simulink model "AcceleratationCore"  (R2024b)
settings: Solver=FixedStepDiscrete  StartTime=0.0  StopTime=inf  FixedStep=1  RelTol=1e-3
model workspace (MATLAB code in the model file):
  | B      = 64;  K = 11;  Cin = 3;
  | L      = 2^nextpow2(B+K-1);   LOG2L = log2(L);   LOG2B = log2(B);
  | NKEEP  = L/2 + 1;
  | LAT    = 307;                              % from FFT_core icon after Ctrl+D
  | W      = ceil((LAT - L + NKEEP + 1)/L);    % wait frames
  | NFR    = B + W + NKEEP;                    % frames per channel
  | PH_W   = ceil(log2(NFR*L));   F_W = PH_W - LOG2L;
  | OC_MAX = (B + NKEEP)*L - 1;   OC_W = ceil(log2(OC_MAX + 1));
  | RAM_AW = LOG2B + LOG2L - 1;
  | WL_BUF = 16;
  | root = fileparts(get_param('AcceleratationCore', 'FileName'));            % repo root = first parent with "vectors"
  | while ~isfolder(fullfile(root, 'vectors')), up = fileparts(root); assert(~strcmp(up, root), 'Repo root not found.'); root = up; end
  | IMG = imresize(imread(fullfile(root, 'resources', 'fujian_mountain_227.png')), [227 227]);   % 227x227x3 uint8
  | Wk  = load(fullfile(root, 'vectors', 'phase1_inputs.mat'), 'W');
  | TILE = IMG(1:B, 1:B, 1);                       % first tile, R channel
  | P = zeros(ceil(size(IMG,1)/B)*B, ceil(size(IMG,2)/B)*B, 3, 'uint8');  P(1:size(IMG,1), 1:size(IMG,2), :) = IMG;
  | IMG_VEC = reshape(permute(reshape(P, B, size(P,1)/B, B, size(P,2)/B, 3), [3 1 5 4 2]), [], 1);   % tiles x Cin x B^2
  | TILE_VEC = reshape(TILE.', [], 1);             % row-major, as will send
  | Cout    = 2;                                   % first test, back to 96 after
  | X_WL    = 2*LOG2B + 8 + 1;                     % B*B*255 < 2^(X_WL-1)
  | KERN_WL = 16;                                  % kernel word (16-bit SDRAM)
  | ACC_WL  = X_WL + KERN_WL + 1 + ceil(log2(Cin));
  | TILE3_VEC = reshape(permute(IMG(1:B, 1:B, :), [2 1 3]), [], 1);   % 3 channels, row-major
  | Hk = fft2(rot90(Wk.W(:, :, :, 1:Cout), 2), L, L) / 255;          % Phase 1 method, 1/255 folded
  | Hk = Hk(:, 1:NKEEP, :, :);                                       % Hermitian half
  | s  = KERN_WL - 2 - floor(log2(max(abs([real(Hk(:)); imag(Hk(:))]))));
  | KERN_TAB = int16(round(reshape(permute(Hk, [3 1 2 4]), Cin, []) * 2^s));
  | IF_WL = 18;   % ifft2d datapath word length (18x18 DSP mode)
  | D_IN  = 16;   % measured 15 on fujian tile 1 (Cout 96) + 1 bit margin; saturation guards outliers
  | D_MID = 4;    % measured 3 + 1 bit margin
  | clear Wk
libraries: hdlsllib x5
settings Model: SimulationMode=accelerator  NumberOfSteps=100  Creator=aaala  LastModifiedBy=aaala
settings OptimizationCC: BlockReduction=off  ConditionallyExecuteInputs=off  DefaultParameterBehavior=Inlined
settings DebuggingCC: AlgebraicLoopMsg=error  InheritedTsInSrcMsg=error
settings HardwareCC: ProdBitPerPointer=32  ProdBitPerSizeT=32  ProdBitPerPtrDiffT=32  ProdLargestAtomicFloat=None  ProdIntDivRoundTo=Undefined  ProdEndianess=Unspecified  ProdWordSize=32  ProdHWDeviceType=ASIC/FPGA->ASIC/FPGA  TargetBitPerPointer=64  TargetBitPerSizeT=64  TargetBitPerPtrDiffT=64  TargetLongLongMode=on  TargetIntDivRoundTo=Zero  TargetEndianess=LittleEndian  TargetWordSize=64  TargetHWDeviceType=Custom Processor->MATLAB Host Computer  ProdEqTarget=off

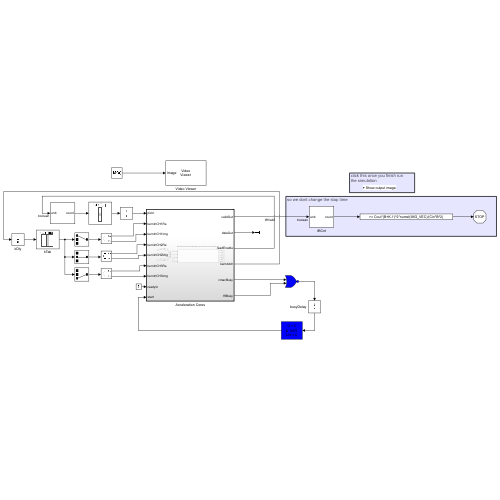
[thumbnail: Simulink's stored preview of the top-level diagram]
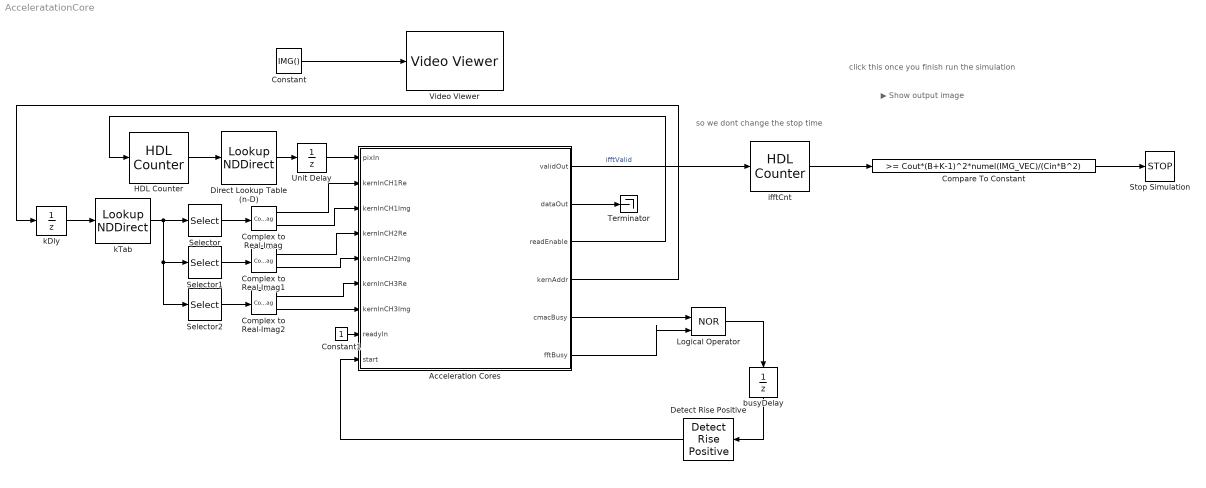
== system AcceleratationCore ==
  note: so we dont change the stop time
  note: ▶ Show output image
  note: click this once you finish run
      | the simulation
  Acceleration Cores : Subsystem  TreatAsAtomicUnit=on
  Compare To Constant : hdlsllib/Logic and Bit Operations/Compare To Constant  relop=>=  const=Cout*(B+K-1)^2*numel(IMG_VEC)/(Cin*B^2)  OutDataTypeStr=boolean
  Complex to Real-Imag : ComplexToRealImag
  Complex to Real-Imag1 : ComplexToRealImag
  Complex to Real-Imag2 : ComplexToRealImag
  Constant : Constant  Value=IMG()  OutDataTypeStr=uint8
  Constant1 : Constant  OutDataTypeStr=boolean
  Detect Rise Positive : hdlsllib/Logic and Bit Operations/Detect Rise Positive  vinit=0  OutDataTypeStr=boolean
  Direct Lookup Table (n-D) : LookupNDDirect  NumberOfTableDimensions=1  Table=IMG_VEC  DiagnosticForOutOfRangeInput=Error
  HDL Counter : hdlsllib/Sources/HDL Counter  CountType=Count limited  CountInit=0  CountStep=1  CountMax=numel(IMG_VEC)-1  CountFromType=Initial value  CountFrom=0  CountResetPort=off  CountLoadPort=off  CountEnbPort=on  CountDirPort=off  CountHitOutputPort=off  CountDataType=Unsigned  CountWordLen=18  CountFracLen=0  CountSampTime=1
  Logical Operator : Logic  Operator=NOR  IconShape=distinctive  AllPortsSameDT=off  OutDataTypeStr=boolean
  Selector : Selector  InputPortWidth=3  IndexOptions=Index vector (dialog)  Indices=[1]  OutputSizes=1
  Selector1 : Selector  InputPortWidth=3  IndexOptions=Index vector (dialog)  Indices=[2]  OutputSizes=1
  Selector2 : Selector  InputPortWidth=3  IndexOptions=Index vector (dialog)  Indices=[3]  OutputSizes=1
  Stop Simulation : Stop
  Terminator : Terminator
  Unit Delay : UnitDelay  SampleTime=-1  HasFrameUpgradeWarning=on
  Video Viewer : VideoViewer  FigPos=[637 623 368 288]
  busyDelay : UnitDelay  SampleTime=-1  HasFrameUpgradeWarning=on
  ifftCnt : hdlsllib/Sources/HDL Counter  CountType=Free running  CountInit=0  CountStep=1  CountMax=25  CountFromType=Initial value  CountFrom=0  CountResetPort=off  CountLoadPort=off  CountEnbPort=on  CountDirPort=off  CountHitOutputPort=off  CountDataType=Unsigned  CountWordLen=32  CountFracLen=0  CountSampTime=1
  kDly : UnitDelay  SampleTime=-1  HasFrameUpgradeWarning=on
  kTab : LookupNDDirect  InputsSelectThisObjectFromTable=Vector  Table=KERN_TAB  DiagnosticForOutOfRangeInput=Error
  wires:
  Acceleration Cores/2(dataOut) -> Terminator/1
  Acceleration Cores/1(validOut) -> ifftCnt/1  "ifftValid"
  Acceleration Cores/3(readEnable) -> HDL Counter/1
  Constant/1 -> Video Viewer/1
  Direct Lookup Table (n-D)/1 -> Unit Delay/1
  Compare To Constant/1 -> Stop Simulation/1
  HDL Counter/1 -> Direct Lookup Table (n-D)/1
  Unit Delay/1 -> Acceleration Cores/1(pixIn)
  ifftCnt/1 -> Compare To Constant/1
  kDly/1 -> kTab/1
  Logical Operator/1 -> busyDelay/1
  Acceleration Cores/4(kernAddr) -> kDly/1
  Constant1/1 -> Acceleration Cores/8(readyIn)
  Detect Rise Positive/1 -> Acceleration Cores/9(start)
  Acceleration Cores/5(cmacBusy) -> Logical Operator/1
  Acceleration Cores/6(fftBusy) -> Logical Operator/2
  busyDelay/1 -> Detect Rise Positive/1
  kTab/1 -> Selector2/1, Selector1/1, Selector/1
  Selector/1 -> Complex to Real-Imag/1
  Selector1/1 -> Complex to Real-Imag1/1
  Selector2/1 -> Complex to Real-Imag2/1
  Complex to Real-Imag/1 -> Acceleration Cores/2(kernInCH1Re)
  Complex to Real-Imag/2 -> Acceleration Cores/3(kernInCH1Img)
  Complex to Real-Imag1/1 -> Acceleration Cores/4(kernInCH2Re)
  Complex to Real-Imag1/2 -> Acceleration Cores/5(kernInCH2Img)
  Complex to Real-Imag2/1 -> Acceleration Cores/6(kernInCH3Re)
  Complex to Real-Imag2/2 -> Acceleration Cores/7(kernInCH3Img)

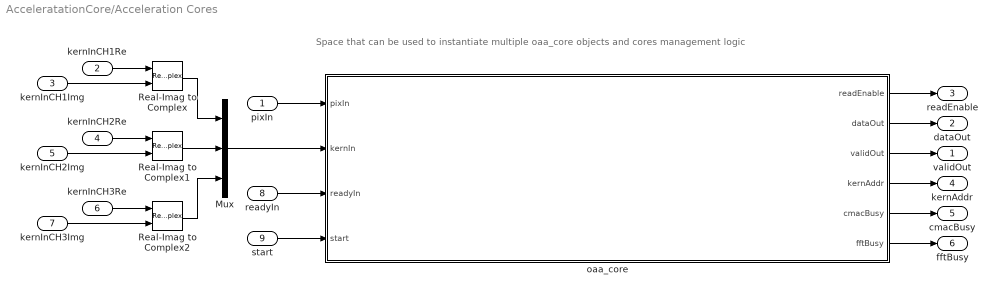
== system AcceleratationCore/Acceleration Cores ==
  note: Space that can be used to instantiate multiple oaa_core objects and cores management logic
  pixIn : Inport
  kernInCH1Re : Inport  Port=2
  kernInCH1Img : Inport  Port=3
  kernInCH2Re : Inport  Port=4
  kernInCH2Img : Inport  Port=5
  kernInCH3Re : Inport  Port=6
  kernInCH3Img : Inport  Port=7
  readyIn : Inport  Port=8
  start : Inport  Port=9
  Mux : Mux  Inputs=3
  Real-Imag to Complex : RealImagToComplex
  Real-Imag to Complex1 : RealImagToComplex
  Real-Imag to Complex2 : RealImagToComplex
  "oaa_core " : Subsystem
  validOut : Outport
  dataOut : Outport  Port=2
  readEnable : Outport  Port=3
  kernAddr : Outport  Port=4
  cmacBusy : Outport  Port=5
  fftBusy : Outport  Port=6
  wires:
  "oaa_core "/3(validOut) -> validOut/1
  "oaa_core "/2(dataOut) -> dataOut/1
  "oaa_core "/1(readEnable) -> readEnable/1
  pixIn/1 -> "oaa_core "/1(pixIn)
  "oaa_core "/4(kernAddr) -> kernAddr/1
  readyIn/1 -> "oaa_core "/3(readyIn)
  start/1 -> "oaa_core "/4(start)
  "oaa_core "/5(cmacBusy) -> cmacBusy/1
  "oaa_core "/6(fftBusy) -> fftBusy/1
  kernInCH1Re/1 -> Real-Imag to Complex/1
  kernInCH1Img/1 -> Real-Imag to Complex/2
  kernInCH2Re/1 -> Real-Imag to Complex1/1
  kernInCH2Img/1 -> Real-Imag to Complex1/2
  kernInCH3Re/1 -> Real-Imag to Complex2/1
  kernInCH3Img/1 -> Real-Imag to Complex2/2
  Real-Imag to Complex/1 -> Mux/1
  Real-Imag to Complex1/1 -> Mux/2
  Real-Imag to Complex2/1 -> Mux/3
  Mux/1 -> "oaa_core "/2(kernIn)

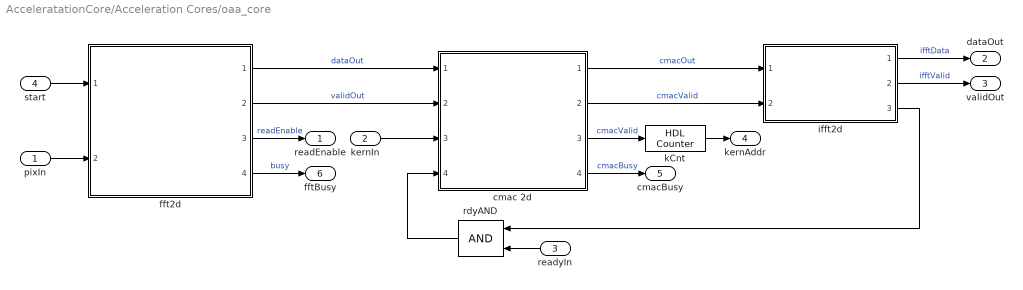
== system AcceleratationCore/Acceleration Cores/oaa_core  ==
  pixIn : Inport
  kernIn : Inport  Port=2
  readyIn : Inport  Port=3
  start : Inport  Port=4
  cmac 2d : Subsystem  ReferencedSubsystem=cmac2d
  "fft2d " : Subsystem  ReferencedSubsystem=fft2d
  ifft2d : Subsystem  ReferencedSubsystem=ifft2d
  kCnt : hdlsllib/Sources/HDL Counter  CountType=Count limited  CountInit=0  CountStep=1  CountMax=size(KERN_TAB,2)-1  CountFromType=Initial value  CountFrom=0  CountResetPort=off  CountLoadPort=off  CountEnbPort=on  CountDirPort=off  CountHitOutputPort=off  CountDataType=Unsigned  CountWordLen=ceil(log2(Cout*L*NKEEP))  CountFracLen=0  CountSampTime=1
  rdyAND : Logic  IconShape=distinctive  AllPortsSameDT=off  OutDataTypeStr=boolean
  readEnable : Outport
  dataOut : Outport  Port=2
  validOut : Outport  Port=3
  kernAddr : Outport  Port=4
  cmacBusy : Outport  Port=5
  fftBusy : Outport  Port=6
  wires:
  start/1 -> "fft2d "/1
  pixIn/1 -> "fft2d "/2
  readyIn/1 -> rdyAND/2
  kernIn/1 -> cmac 2d/3
  "fft2d "/1 -> cmac 2d/1  "dataOut"
  "fft2d "/2 -> cmac 2d/2  "validOut"
  "fft2d "/3 -> readEnable/1  "readEnable"
  "fft2d "/4 -> fftBusy/1  "busy"
  rdyAND/1 -> cmac 2d/4
  cmac 2d/2 -> ifft2d/2  "cmacValid"
  cmac 2d/1 -> ifft2d/1  "cmacOut"
  cmac 2d/4 -> cmacBusy/1  "cmacBusy"
  ifft2d/2 -> validOut/1  "ifftValid"
  ifft2d/1 -> dataOut/1  "ifftData"
  ifft2d/3 -> rdyAND/1
  kCnt/1 -> kernAddr/1
  cmac 2d/3 -> kCnt/1  "cmacValid"
